simulink model "lab11"  (R2025b)
settings: Solver=VariableStepAuto  StartTime=0.0  StopTime=10.0  RelTol=1e-3
undefined symbols (not defined in the file): A, b, gamma, K, P
settings Model: Creator=Nickolay  LastModifiedBy=Nickolay

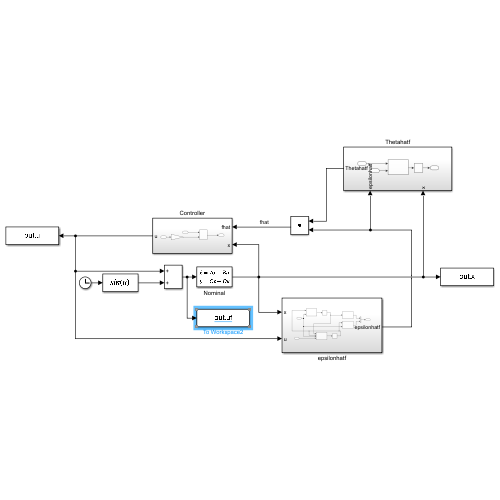
[thumbnail: Simulink's stored preview of the top-level diagram]
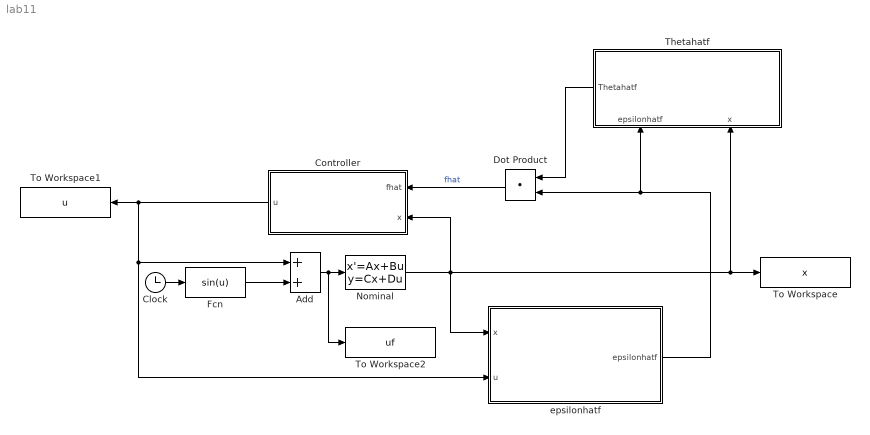
== system lab11 ==
  Add : Sum
  Clock : Clock
  Controller : Subsystem
  Dot Product : DotProduct  OutDataTypeStr=Inherit: Inherit via internal rule
  Fcn : Fcn  Expr=sin(u)
  Nominal : StateSpace  A=A  B=b  C=eye(2)  D=zeros(2,1)  InitialCondition=0
  Thetahatf : Subsystem
      settings: PortSchema="{\"entries\":[{\"content\":{\"sides\":[{\"content\":{},\"type\":\"ConnectorPlacement.EquallySpacedRectSide\",\"uuid\":\"ae71786c-eb3f-40eb-98a9-01c665788276\"},{\"content\":{\"connectorIds\":[\"Out1\"],\"side\":\"RIGHT\"},\"type\":\"ConnectorPlacement.EquallySpacedRectSide\",\"uuid\":\"271eaff9-e73d-48b6-a569-2ebd70f67efd\"},{\"content\":{\"side\":\"TOP\"},\"type\":\"ConnectorPlacement.EquallySpacedRectSide\",\"uuid\":\"0d499bdb-c0c5-4154-8767-1f41a00543b0\"},{\"content\":{\"connectorIds\":[\"In1\",\"In2\"],\"side\":\"BOTTOM\"},\"type\":\"ConnectorPlacement.EquallySpacedRectSide\",\"uuid\":\"ac53d6df-f3dc-44d0-a43d-62807c6aa5e3\"}]},\"type\":\"ConnectorPlacement.EquallySpacedConnector\",\"uuid\":\"bdae0fc1-a417-4268-a6b2-1e71d02ed00d\"}],\"packageUris\":[\"http://schema.mathworks.com/mf0/Connector/R2020b\"],\"version\":\"1.0\"}"
  To Workspace : ToWorkspace  VariableName=x  SaveFormat=Timeseries  SampleTime=-1
  To Workspace1 : ToWorkspace  VariableName=u  SaveFormat=Timeseries  SampleTime=-1
  To Workspace2 : ToWorkspace  VariableName=uf  SaveFormat=Timeseries  SampleTime=-1
  epsilonhatf : Subsystem
  wires:
  Controller/1(u) -> To Workspace1/1, epsilonhatf/2(u), Add/1
  Nominal/1 -> Controller/2(x), To Workspace/1, Thetahatf/1(x), epsilonhatf/1(x)
  Thetahatf/1(Thetahatf) -> Dot Product/1
  epsilonhatf/1(epsilonhatf) -> Thetahatf/2(epsilonhatf), Dot Product/2
  Dot Product/1 -> Controller/1(fhat)  "fhat"
  Add/1 -> To Workspace2/1, Nominal/1
  Clock/1 -> Fcn/1
  Fcn/1 -> Add/2

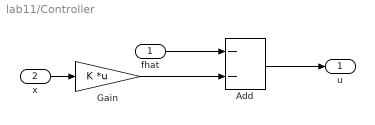
== system lab11/Controller ==
  fhat : Inport
  x : Inport  Port=2
  Add : Sum  Inputs=--
  Gain : Gain  Gain=K  Multiplication=Matrix(K*u) (u vector)
  u : Outport
  wires:
  fhat/1 -> Add/1
  Add/1 -> u/1
  x/1 -> Gain/1
  Gain/1 -> Add/2

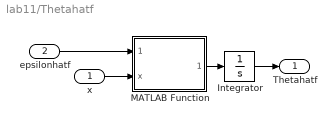
== system lab11/Thetahatf ==
  x : Inport
  epsilonhatf : Inport  Port=2
  Integrator : Integrator  InitialCondition=[0;0]
  MATLAB Function : MATLAB Function  TreatAsAtomicUnit=on
  Thetahatf : Outport
  wires:
  epsilonhatf/1 -> MATLAB Function/1(epsilonhatf)
  x/1 -> MATLAB Function/2(x)
  Integrator/1 -> Thetahatf/1
  MATLAB Function/1(thetahatfder) -> Integrator/1

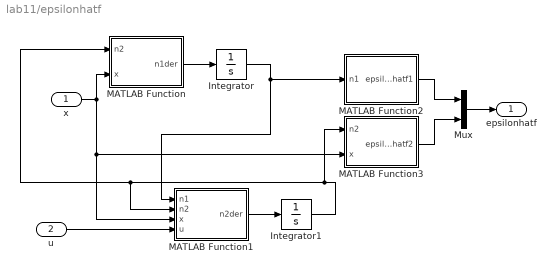
== system lab11/epsilonhatf ==
  x : Inport
  u : Inport  Port=2
  Integrator : Integrator
  Integrator1 : Integrator
  MATLAB Function : MATLAB Function  TreatAsAtomicUnit=on
  MATLAB Function1 : MATLAB Function  TreatAsAtomicUnit=on
  MATLAB Function2 : MATLAB Function  TreatAsAtomicUnit=on
  MATLAB Function3 : MATLAB Function  TreatAsAtomicUnit=on
  Mux : Mux  Inputs=2
  epsilonhatf : Outport
  wires:
  MATLAB Function/1(n1der) -> Integrator/1
  Integrator1/1 -> MATLAB Function3/1(n2), MATLAB Function/1(n2), MATLAB Function1/2(n2)
  MATLAB Function1/1(n2der) -> Integrator1/1
  x/1 -> MATLAB Function3/2(x), MATLAB Function1/3(x), MATLAB Function/2(x)
  u/1 -> MATLAB Function1/4(u)
  Integrator/1 -> MATLAB Function2/1(n1), MATLAB Function1/1(n1)
  MATLAB Function2/1(epsilonhatf1) -> Mux/1
  MATLAB Function3/1(epsilonhatf2) -> Mux/2
  Mux/1 -> epsilonhatf/1

== matlab function lab11/epsilonhatf/MATLAB Function1 ==
  data: n1 input; n2 input; n2der output; x input; u input
function n2der = fcn(n1, n2, x, u)
n2der = -0.01*n1-0.2*n2-1.04*x(1)-0.68*x(2)-u;

== matlab function lab11/epsilonhatf/MATLAB Function ==
  data: n2 input; n1der output; x input
function n1der = fcn(n2, x)
n1der = n2+0.2*x(1)+0.4*x(2);

== matlab function lab11/epsilonhatf/MATLAB Function2 ==
  data: n1 input; epsilonhatf1 output
function epsilonhatf1 = fcn(n1)
epsilonhatf1 = n1;

== matlab function lab11/epsilonhatf/MATLAB Function3 ==
  data: n2 input; epsilonhatf2 output; x input
function epsilonhatf2 = fcn(n2, x)
epsilonhatf2 = n2 + 0.2*x(1) + 0.4*x(2);

== matlab function lab11/Thetahatf/MATLAB Function ==
  data: epsilonhatf input; thetahatfder output; x input; gamma parameter; b parameter; P parameter
function thetahatfder = fcn(epsilonhatf, x, gamma, b, P)

thetahatfder = gamma*epsilonhatf*b.'*P*x;
